simulink model "Test_Sensors"  (R2026a)
settings: Solver=FixedStepAuto  StopTime=20  FixedStep=SIM.FixedStepSize
undefined symbols (not defined in the file): SIM
settings Model: Creator=emrec  LastModifiedBy=emrec
settings DebuggingCC: InheritedTsInSrcMsg=none

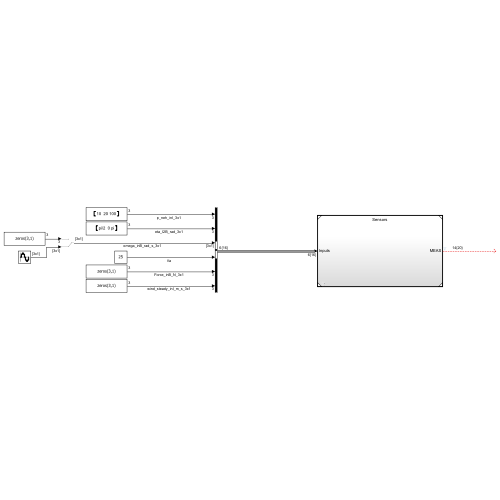
[thumbnail: Simulink's stored preview of the top-level diagram]
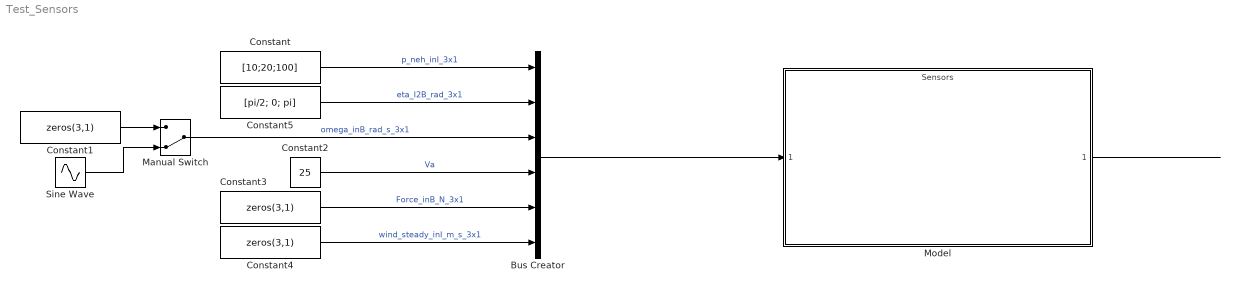
== system Test_Sensors ==
  Bus Creator : BusCreator  Inputs=6  OutDataTypeStr=Bus: SensorsInputsBus
      settings: InheritFromInputs=off
  Constant : Constant  Value=[10;20;100]
  Constant1 : Constant  Value=zeros(3,1)
  Constant2 : Constant  Value=25
  Constant3 : Constant  Value=zeros(3,1)
  Constant4 : Constant  Value=zeros(3,1)
  Constant5 : Constant  Value=[pi/2; 0; pi]
  Manual Switch : ManualSwitch  CurrentSetting=0
  Model : ModelReference  ModelNameDialog=Sensors.slx  SimulationMode=Normal  ModelReferenceVersion=1.11
  Sine Wave : Sin  Amplitude=pi  Frequency=2*pi * 0.5  Phase=[0; -2*pi/3; 2*pi/3]  SampleTime=SIM.FixedStepSize  VectorParams1D=off
  wires:
  Bus Creator/1 -> Model/1
  Constant/1 -> Bus Creator/1  "p_neh_inI_3x1"
  Constant5/1 -> Bus Creator/2  "eta_I2B_rad_3x1"
  Constant1/1 -> Manual Switch/1
  Constant2/1 -> Bus Creator/4  "Va"
  Constant3/1 -> Bus Creator/5  "Force_inB_N_3x1"
  Constant4/1 -> Bus Creator/6  "wind_steady_inI_m_s_3x1"
  Model/1 -> ?
  Manual Switch/1 -> Bus Creator/3  "omega_inB_rad_s_3x1"
  Sine Wave/1 -> Manual Switch/2
